simulink model "FDIR_SensorFault_Subsystem_2026a"  (R2026a)
settings: Solver=VariableStepAuto
settings Model: Creator=jayby  LastModifiedBy=aditi
settings SFSimCC: SimGPUStackLimitPerThread=51200
settings RTWCC: GPUStackLimitPerThread=51200

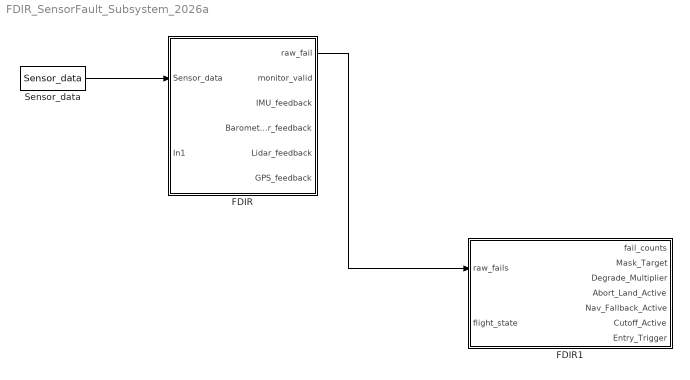
== system FDIR_SensorFault_Subsystem_2026a ==
  FDIR : Subsystem
  FDIR1 : Subsystem
  Sensor_data : FromWorkspace  VariableName=Sensor_data
  wires:
  Sensor_data/1 -> FDIR/1(Sensor_data)
  FDIR/1(raw_fail) -> FDIR1/1(raw_fails)

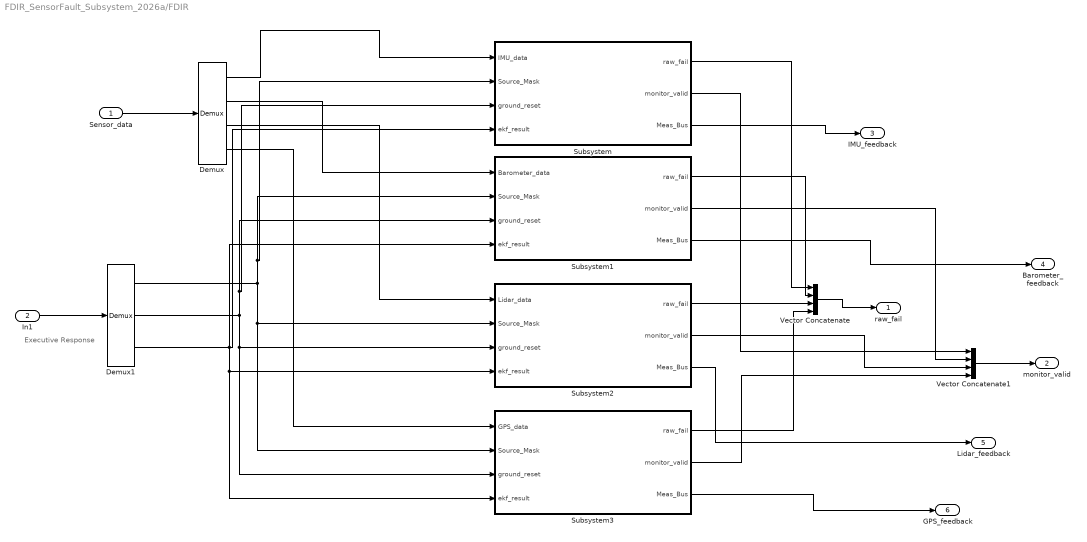
== system FDIR_SensorFault_Subsystem_2026a/FDIR ==
  note: Executive Response
  Sensor_data : Inport
  In1 : Inport  Port=2
  Demux : Demux
  Demux1 : Demux  Outputs=3
  Subsystem : Subsystem
  Subsystem1 : Subsystem
  Subsystem2 : Subsystem
  Subsystem3 : Subsystem
  Vector Concatenate : Concatenate  NumInputs=4
  Vector Concatenate1 : Concatenate  NumInputs=4
  raw_fail : Outport
  monitor_valid : Outport  Port=2
  IMU_feedback : Outport  Port=3
  Barometer_feedback : Outport  Port=4
  Lidar_feedback : Outport  Port=5
  GPS_feedback : Outport  Port=6
  wires:
  Sensor_data/1 -> Demux/1
  Demux/1 -> Subsystem/1(IMU_data)
  Demux/2 -> Subsystem1/1(Barometer_data)
  Demux/3 -> Subsystem2/1(Lidar_data)
  Demux/4 -> Subsystem3/1(GPS_data)
  In1/1 -> Demux1/1
  Demux1/1 -> Subsystem1/2(Source_Mask), Subsystem/2(Source_Mask), Subsystem3/2(Source_Mask), Subsystem2/2(Source_Mask)
  Demux1/2 -> Subsystem1/3(ground_reset), Subsystem/3(ground_reset), Subsystem3/3(ground_reset), Subsystem2/3(ground_reset)
  Demux1/3 -> Subsystem3/4(ekf_result), Subsystem2/4(ekf_result), Subsystem1/4(ekf_result), Subsystem/4(ekf_result)
  Subsystem/1(raw_fail) -> Vector Concatenate/1
  Subsystem1/1(raw_fail) -> Vector Concatenate/2
  Subsystem2/1(raw_fail) -> Vector Concatenate/3
  Subsystem3/1(raw_fail) -> Vector Concatenate/4
  Vector Concatenate/1 -> raw_fail/1
  Vector Concatenate1/1 -> monitor_valid/1
  Subsystem3/2(monitor_valid) -> Vector Concatenate1/4
  Subsystem1/2(monitor_valid) -> Vector Concatenate1/2
  Subsystem2/2(monitor_valid) -> Vector Concatenate1/3
  Subsystem/2(monitor_valid) -> Vector Concatenate1/1
  Subsystem/3(Meas_Bus) -> IMU_feedback/1
  Subsystem1/3(Meas_Bus) -> Barometer_feedback/1
  Subsystem2/3(Meas_Bus) -> Lidar_feedback/1
  Subsystem3/3(Meas_Bus) -> GPS_feedback/1

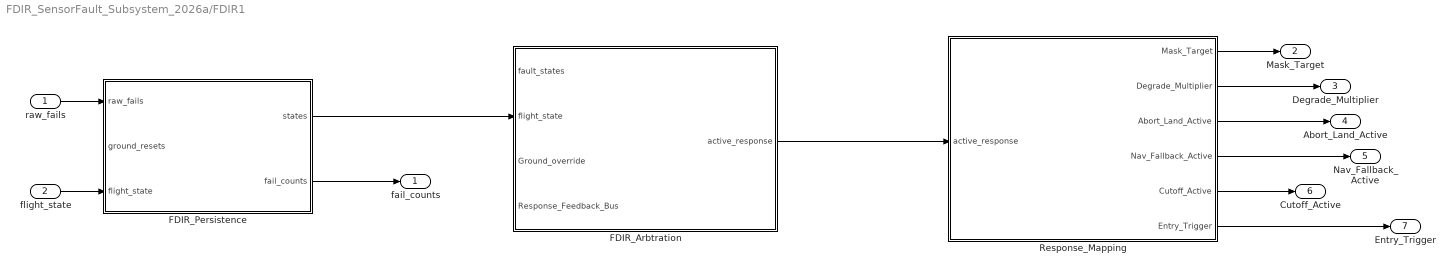
== system FDIR_SensorFault_Subsystem_2026a/FDIR1 ==
  raw_fails : Inport
  flight_state : Inport  Port=2
  FDIR_Arbtration : MATLAB Function  TreatAsAtomicUnit=on
  FDIR_Persistence : MATLAB Function  TreatAsAtomicUnit=on
  Response_Mapping : MATLAB Function  TreatAsAtomicUnit=on
  fail_counts : Outport
  Mask_Target : Outport  Port=2
  Degrade_Multiplier : Outport  Port=3
  Abort_Land_Active : Outport  Port=4
  Nav_Fallback_Active : Outport  Port=5
  Cutoff_Active : Outport  Port=6
  Entry_Trigger : Outport  Port=7
  wires:
  raw_fails/1 -> FDIR_Persistence/1(raw_fails)
  flight_state/1 -> FDIR_Persistence/3(flight_state)
  FDIR_Persistence/1(states) -> FDIR_Arbtration/2(flight_state)
  FDIR_Arbtration/1(active_response) -> Response_Mapping/1(active_response)
  FDIR_Persistence/2(fail_counts) -> fail_counts/1
  Response_Mapping/1(Mask_Target) -> Mask_Target/1
  Response_Mapping/2(Degrade_Multiplier) -> Degrade_Multiplier/1
  Response_Mapping/3(Abort_Land_Active) -> Abort_Land_Active/1
  Response_Mapping/4(Nav_Fallback_Active) -> Nav_Fallback_Active/1
  Response_Mapping/5(Cutoff_Active) -> Cutoff_Active/1
  Response_Mapping/6(Entry_Trigger) -> Entry_Trigger/1

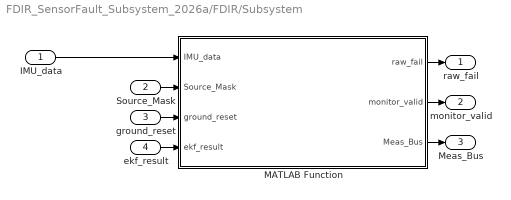
== system FDIR_SensorFault_Subsystem_2026a/FDIR/Subsystem ==
  IMU_data : Inport
  Source_Mask : Inport  Port=2
  ground_reset : Inport  Port=3
  ekf_result : Inport  Port=4
  MATLAB Function : MATLAB Function  TreatAsAtomicUnit=on
  raw_fail : Outport
  monitor_valid : Outport  Port=2
  Meas_Bus : Outport  Port=3
  wires:
  ground_reset/1 -> MATLAB Function/3(ground_reset)
  Source_Mask/1 -> MATLAB Function/2(Source_Mask)
  MATLAB Function/2(monitor_valid) -> monitor_valid/1
  MATLAB Function/3(Meas_Bus) -> Meas_Bus/1
  ekf_result/1 -> MATLAB Function/4(ekf_result)
  MATLAB Function/1(raw_fail) -> raw_fail/1
  IMU_data/1 -> MATLAB Function/1(IMU_data)

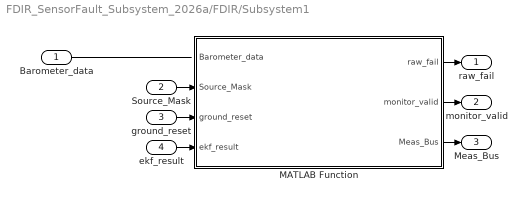
== system FDIR_SensorFault_Subsystem_2026a/FDIR/Subsystem1 ==
  Barometer_data : Inport
  Source_Mask : Inport  Port=2
  ground_reset : Inport  Port=3
  ekf_result : Inport  Port=4
  MATLAB Function : MATLAB Function  TreatAsAtomicUnit=on
  raw_fail : Outport
  monitor_valid : Outport  Port=2
  Meas_Bus : Outport  Port=3
  wires:
  ground_reset/1 -> MATLAB Function/3(ground_reset)
  Source_Mask/1 -> MATLAB Function/2(Source_Mask)
  MATLAB Function/2(monitor_valid) -> monitor_valid/1
  MATLAB Function/3(Meas_Bus) -> Meas_Bus/1
  ekf_result/1 -> MATLAB Function/4(ekf_result)
  MATLAB Function/1(raw_fail) -> raw_fail/1
  Barometer_data/1 -> ?

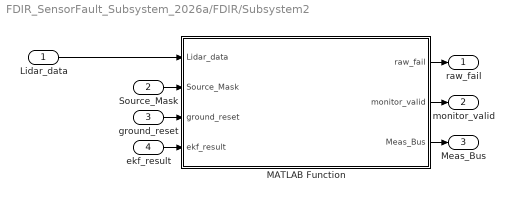
== system FDIR_SensorFault_Subsystem_2026a/FDIR/Subsystem2 ==
  Lidar_data : Inport
  Source_Mask : Inport  Port=2
  ground_reset : Inport  Port=3
  ekf_result : Inport  Port=4
  MATLAB Function : MATLAB Function  TreatAsAtomicUnit=on
  raw_fail : Outport
  monitor_valid : Outport  Port=2
  Meas_Bus : Outport  Port=3
  wires:
  ground_reset/1 -> MATLAB Function/3(ground_reset)
  Source_Mask/1 -> MATLAB Function/2(Source_Mask)
  MATLAB Function/2(monitor_valid) -> monitor_valid/1
  MATLAB Function/3(Meas_Bus) -> Meas_Bus/1
  ekf_result/1 -> MATLAB Function/4(ekf_result)
  MATLAB Function/1(raw_fail) -> raw_fail/1
  Lidar_data/1 -> MATLAB Function/1(Lidar_data)

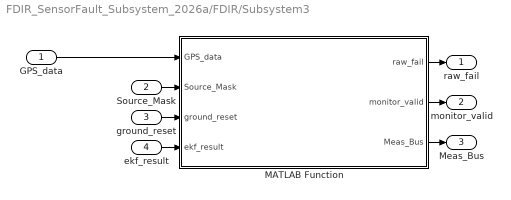
== system FDIR_SensorFault_Subsystem_2026a/FDIR/Subsystem3 ==
  GPS_data : Inport
  Source_Mask : Inport  Port=2
  ground_reset : Inport  Port=3
  ekf_result : Inport  Port=4
  MATLAB Function : MATLAB Function  TreatAsAtomicUnit=on
  raw_fail : Outport
  monitor_valid : Outport  Port=2
  Meas_Bus : Outport  Port=3
  wires:
  ground_reset/1 -> MATLAB Function/3(ground_reset)
  Source_Mask/1 -> MATLAB Function/2(Source_Mask)
  MATLAB Function/2(monitor_valid) -> monitor_valid/1
  MATLAB Function/3(Meas_Bus) -> Meas_Bus/1
  ekf_result/1 -> MATLAB Function/4(ekf_result)
  MATLAB Function/1(raw_fail) -> raw_fail/1
  GPS_data/1 -> MATLAB Function/1(GPS_data)

== matlab function FDIR_SensorFault_Subsystem_2026a/FDIR1/FDIR_Arbtration ==
  data: fault_states input; active_response output; flight_state input; Ground_override input; Response_Feedback_Bus input
function active_response = fdir_arbitration(fault_states, flight_state, Ground_override, Response_Feedback_Bus)
persistent current_response;

if isempty(current_response)
    current_response = uint8(0); % R0 (Nominal)
end

LANDED_PHASE = uint8(5);

% Allow reset only on ground with override active
if Ground_override && (flight_state == LANDED_PHASE)
    current_response = uint8(0);
    active_response = current_response;
    return;
end

max_requested = uint8(0);

for i = 1:length(fault_states)
    sensor_state = fault_states(i).Persistence_State;

    % If fault is latched (state == 2), query its response tier from fault_config
    if sensor_state == uint8(2)
        req = fault_config(i).Response_Tier;
    else
        req = uint8(0);
    end

    if req > max_requested
        max_requested = req;
    end
end

% Latch highest escalation level (prevent dropping back down mid-flight)
if max_requested > current_response
    current_response = max_requested;
end

active_response = current_response;
end

== matlab function FDIR_SensorFault_Subsystem_2026a/FDIR1/FDIR_Persistence ==
  data: raw_fails input; states output; ground_resets input; flight_state input; fail_counts output
function [states, fail_counts] = fdir_persistence(raw_fails, ground_resets, flight_state)
% Dynamic N-of-M Persistence Filter for all fault monitors
persistent history;     
persistent states_vec;  
persistent first_timestamps;
persistent sim_time;

M = 10; % Rolling window size
N = 4;  % Failure threshold

active_phases = [2, 3, 4]; % Active flight phases (e.g., Ascent, Burn)
num_faults = length(raw_fails);

if isempty(history)
    history = false(num_faults, M);
    states_vec = zeros(num_faults, 1, 'uint8');
    first_timestamps = zeros(num_faults, 1);
    sim_time = 0.0;
end

sim_time = sim_time + 0.01; % 100 Hz frame rate increment
fail_counts = zeros(num_faults, 1, 'uint8');

% Initialize output bus struct template matching Fault_State_Bus
single_fault_struct = struct(...
    'Fault_ID', uint8(0), ...
    'Monitor_Valid', true, ...
    'Raw_Fail', false, ...
    'Persistence_State', uint8(0), ...
    'Fail_Count', uint8(0), ...
    'First_Fault_Timestamp', 0.0 ...
    );
states = repmat(single_fault_struct, num_faults, 1);

for i = 1:num_faults
    states(i).Fault_ID = uint8(i);
    states(i).Monitor_Valid = true;
    states(i).Raw_Fail = logical(raw_fails(i));

    % Handle individual Ground Reset
    if ground_resets(i)
        history(i, :) = false(1, M);
        states_vec(i) = uint8(0);
        fail_counts(i) = uint8(0);
        first_timestamps(i) = 0.0;
        states(i).Persistence_State = states_vec(i);
        states(i).Fail_Count = fail_counts(i);
        states(i).First_Fault_Timestamp = first_timestamps(i);
        continue;
    end

    % Pause evaluation if outside active phases
    if ~ismember(flight_state, active_phases)
        if states_vec(i) ~= uint8(2)
            history(i, :) = false(1, M);
            states_vec(i) = uint8(0);
        end
        fail_counts(i) = uint8(sum(history(i, :)));
        states(i).Persistence_State = states_vec(i);
        states(i).Fail_Count = fail_counts(i);
        states(i).First_Fault_Timestamp = first_timestamps(i);
        continue;
    end

    % Hold state if already latched
    if states_vec(i) == uint8(2)
        fail_counts(i) = uint8(sum(history(i, :)));
        states(i).Persistence_State = states_vec(i);
        states(i).Fail_Count = fail_counts(i);
        states(i).First_Fault_Timestamp = first_timestamps(i);
        continue;
    end

    % Shift rolling window and insert sample
    history(i, :) = [history(i, 2:end), logical(raw_fails(i))];
    fail_counts(i) = uint8(sum(history(i, :)));

    % State transitions
    switch states_vec(i)
        case uint8(0) % INACTIVE
            if raw_fails(i)
                states_vec(i) = uint8(1); % PENDING
                first_timestamps(i) = sim_time;
            end
        case uint8(1) % PENDING
            if fail_counts(i) >= N
                states_vec(i) = uint8(2); % LATCHED
            elseif fail_counts(i) == 0
                states_vec(i) = uint8(0); % INACTIVE
                first_timestamps(i) = 0.0;
            end
        case uint8(2) % LATCHED
            states_vec(i) = uint8(2);
    end

    states(i).Persistence_State = states_vec(i);
    states(i).Fail_Count = fail_counts(i);
    states(i).First_Fault_Timestamp = first_timestamps(i);
end
end

== matlab function FDIR_SensorFault_Subsystem_2026a/FDIR1/Response_Mapping ==
  data: active_response input; Mask_Target output; Degrade_Multiplier output; Abort_Land_Active output; Nav_Fallback_Active output; Cutoff_Active output; Entry_Trigger output
function [Mask_Target, Degrade_Multiplier, Abort_Land_Active, Nav_Fallback_Active, Cutoff_Active, Entry_Trigger] = response_mapping(active_response)
% Maps active response tier (0-4) to subsystem command signals

% Initialize outputs to safe nominal defaults
Mask_Target = false;
Degrade_Multiplier = 1.0;
Abort_Land_Active = false;
Nav_Fallback_Active = false;
Cutoff_Active = false;
Entry_Trigger = false;

switch active_response
    case uint8(0) % R0 - Nominal
        % Defaults remain active

    case uint8(1) % R1 - Reconfiguration / Minor Degradation
        Mask_Target = true;
        Degrade_Multiplier = 0.8;

    case uint8(2) % R2 - Safe Mode / Abort Landing
        Mask_Target = true;
        Degrade_Multiplier = 0.5;
        Abort_Land_Active = true;

    case uint8(3) % R3 - Navigation Fallback / Engine Cutoff
        Mask_Target = true;
        Degrade_Multiplier = 0.0;
        Abort_Land_Active = true;
        Nav_Fallback_Active = true;
        Cutoff_Active = true;

    case uint8(4) % R4 - Emergency Escape / Abort
        Mask_Target = true;
        Degrade_Multiplier = 0.0;
        Abort_Land_Active = true;
        Nav_Fallback_Active = true;
        Cutoff_Active = true;
        Entry_Trigger = true;

    otherwise
        % Default safety fallback
        Mask_Target = true;
        Abort_Land_Active = true;
end
end

== matlab function FDIR_SensorFault_Subsystem_2026a/FDIR/Subsystem/MATLAB Function ==
  data: IMU_data input; Source_Mask input; raw_fail output; monitor_valid output; ground_reset input; Meas_Bus output; ekf_result input
function [raw_fail, monitor_valid, Meas_Bus]= fcn(IMU_data, Source_Mask, ground_reset, ekf_result)
    raw_fail = [];
    sensor_range = [-1, 1]; %saturation range
    if (Source_Mask && ~ground_reset)
        monitor_valid = 0;
        Meas_Bus = NaN;
    end
    %Check for loss of data (F-01)
    if (any(IMU_data == Nan) || any(IMU_data == 0))
        raw_fail(end+1) = 1;
    else
        raw_fail(end+1) = 0;
    end
    %Check for IMU drift or bias (F-02), ekf_result needs to be 6 vector
    if (any(abs(IMU_data-ekf_result)>1, 'all')) %How should I define this?
        raw_fail(end+1) = 1;
    else
        raw_fail(end+1) = 0;
    end
    %Check for Saturation
    if ~(any(IMU_data < sensor_range(1)) && any(IMU_data > sensor_range(0)))
        raw_fail(end+1) = 1;
    else
        raw_fail(end+1) = 0;
    end

== matlab function FDIR_SensorFault_Subsystem_2026a/FDIR/Subsystem1/MATLAB Function ==
  data: Barometer_data input; Source_Mask input; raw_fail output; monitor_valid output; ground_reset input; Meas_Bus output; ekf_result input
function [raw_fail, monitor_valid, Meas_Bus]= fcn(Barometer_data, Source_Mask, ground_reset, ekf_result)
    raw_fail = [];
    sensor_range = [-1, 1]; %saturation range
    if (Source_Mask && ~ground_reset)
        monitor_valid = 0;
        Meas_Bus = NaN;
    end
    %Check for loss of data (F-01)
    if (any(Barometer_data == Nan) || any(Barometer_data == 0))
        raw_fail(end+1) = 1;
    else
        raw_fail(end+1) = 0;
    end
    %Check for IMU drift or bias (F-02), ekf_result needs to be 6 vector
    if (any(abs(Barometer_data-ekf_result)>1, 'all')) %How should I define this?
        raw_fail(end+1) = 1;
    else
        raw_fail(end+1) = 0;
    end
    %Check for Saturation
    if ~(any(Barometer_data < sensor_range(1)) && any(Barometer_data > sensor_range(0)))
        raw_fail(end+1) = 1;
    else
        raw_fail(end+1) = 0;
    end

== matlab function FDIR_SensorFault_Subsystem_2026a/FDIR/Subsystem2/MATLAB Function ==
  data: Lidar_data input; Source_Mask input; raw_fail output; monitor_valid output; ground_reset input; Meas_Bus output; ekf_result input
function [raw_fail, monitor_valid, Meas_Bus]= fcn(Lidar_data, Source_Mask, ground_reset, ekf_result)
    raw_fail = [];
    sensor_range = [-1, 1]; %saturation range
    if (Source_Mask && ~ground_reset)
        monitor_valid = 0;
        Meas_Bus = NaN;
    end
    %Check for loss of data (F-01)
    if (any(Lidar_data == Nan) || any(Lidar_data == 0))
        raw_fail(end+1) = 1;
    else
        raw_fail(end+1) = 0;
    end
    %Check for IMU drift or bias (F-02), ekf_result needs to be 6 vector
    if (any(abs(Lidar_data-ekf_result)>1, 'all')) %How should I define this?
        raw_fail(end+1) = 1;
    else
        raw_fail(end+1) = 0;
    end
    %Check for Saturation
    if ~(any(Lidar_data < sensor_range(1)) && any(Lidar_data > sensor_range(0)))
        raw_fail(end+1) = 1;
    else
        raw_fail(end+1) = 0;
    end

== matlab function FDIR_SensorFault_Subsystem_2026a/FDIR/Subsystem3/MATLAB Function ==
  data: GPS_data input; Source_Mask input; raw_fail output; monitor_valid output; ground_reset input; Meas_Bus output; ekf_result input
function [raw_fail, monitor_valid, Meas_Bus]= fcn(GPS_data, Source_Mask, ground_reset, ekf_result)
    raw_fail = [];
    sensor_range = [-1, 1]; %saturation range
    if (Source_Mask && ~ground_reset)
        monitor_valid = 0;
        Meas_Bus = NaN;
    end
    %Check for loss of data (F-01)
    if (any(GPS_data == Nan) || any(GPS_data == 0))
        raw_fail(end+1) = 1;
    else
        raw_fail(end+1) = 0;
    end
    %Check for GPS drift or bias (F-02), ekf_result needs to be 6 vector
    if (any(abs(GPS_data-ekf_result)>1, 'all')) %How should I define this?
        raw_fail(end+1) = 1;
    else
        raw_fail(end+1) = 0;
    end
    %Check for Saturation
    if ~(any(GPS_data < sensor_range(1)) && any(GPS_data > sensor_range(0)))
        raw_fail(end+1) = 1;
    else
        raw_fail(end+1) = 0;
    end
